simulink model "nmr_marginal_osc"  (R2025b)
settings: Solver=ode45  StartTime=0.0  StopTime=P.Tstop  MaxStep=P.maxStep  RelTol=1e-5
PreLoadFcn:
  | nmr_params
InitFcn:
  | nmr_params
undefined symbols (not defined in the file or in its folder): P
libraries: simulink x2
settings Model: Creator=paul  LastModifiedBy=paul

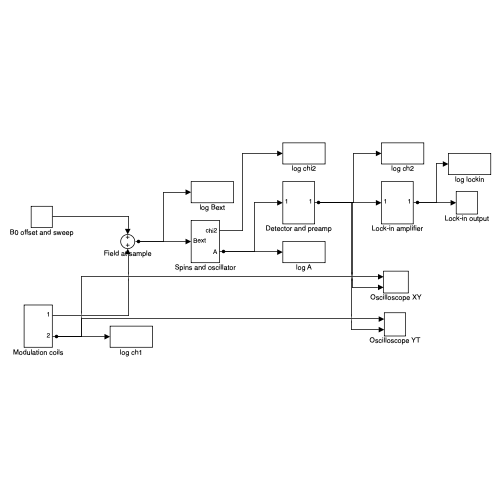
[thumbnail: Simulink's stored preview of the top-level diagram]
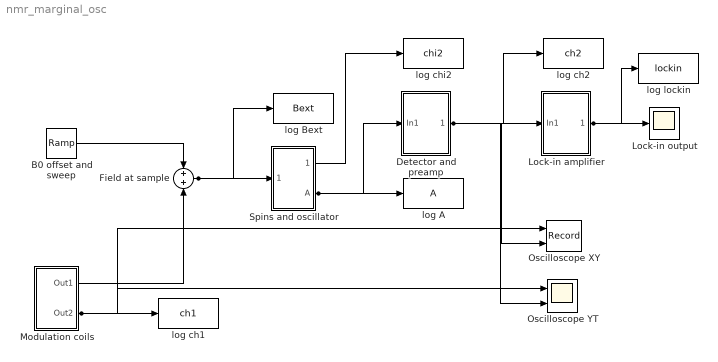
== system nmr_marginal_osc ==
  B0 offset and sweep : simulink/Sources/Ramp  slope=P.sweep  start=0  InitialOutput=P.Boff
  Detector and preamp : Subsystem
  Field at sample : Sum
  Lock-in amplifier : Subsystem
  Lock-in output : Scope
  Modulation coils : Subsystem
  Oscilloscope XY : Record  NumPorts=2.0  FileSettingsInternal="{\"entries\":[{\"content\":{\"excelSettings\":{\"content\":{},\"type\":\"Streamout.ExcelSettings\"},\"parquetSettings\":{\"content\":{},\"type\":\"Streamout.ParquetSettings\"}},\"type\":\"Streamout.FileSettingStorage\",\"uuid\":\"\"}],\"packageUris\":[\"http:\\/\\/schema.mathworks.com\\/mf0\\/streamout_blocks\\/R2020a\"],\"version\":\"1.0\"}"  FrameSettings=[0, 0]  Layout=[1 1]  SignalsInternal="{\"entries\":[{\"content\":{\"signals\":[{\"content\":{\"blockPath\":[],\"dimensions\":[1],\"domain\":\"\",\"lineColor\":\"#a2142f\",\"plots\":[ 1 ],\"port\":1,\"signalID\":1,\"signalName\":\"XY Graph:1\"},\"type\":\"RecordBlkView.Signal\",\"uuid\":\"\"},{\"content\":{\"blockPath\":[],\"dimensions\":[1],\"domain\":\"\",\"lineColor\":\"#139fff\",\"plots\":[ 1 ],\"port\":2,\"signalID\":2,\"signalName\":\"XY Graph:2\"},\"type\":\"RecordBlkView.Signal\",\"uuid\":\"\"}]},\"type\":\"RecordBlkView.InputSignals\",\"uuid\":\"\"}],\"packageUris\":[\"http:\\/\\/schema.mathworks.com\\/mf0\\/streamout_blocks\\/R2020a\"],\"version\":\"1.0\"}"  VisualizationBindings="{\"xyplotplugin\":{\"info\":[{\"series\":[{\"bindingParametersList\":[{\"parameter\":\"X-Axis\",\"signalID\":1,\"signalName\":\"XY Graph:1\"},{\"parameter\":\"Y-Axis\",\"signalID\":2,\"signalName\":\"XY Graph:2\"}],\"seriesID\":0}],\"subplotID\":1}]}}"  CompatibilityTag=XY
  Oscilloscope YT : Scope  NumInputPorts=2
  Spins and oscillator : Subsystem
  log A : ToWorkspace  VariableName=A  SaveFormat=Timeseries  SampleTime=-1
  log Bext : ToWorkspace  VariableName=Bext  SaveFormat=Timeseries  SampleTime=-1
  log ch1 : ToWorkspace  VariableName=ch1  SaveFormat=Timeseries  SampleTime=-1
  log ch2 : ToWorkspace  VariableName=ch2  SaveFormat=Timeseries  SampleTime=-1
  log chi2 : ToWorkspace  VariableName=chi2  SaveFormat=Timeseries  SampleTime=-1
  log lockin : ToWorkspace  VariableName=lockin  SaveFormat=Timeseries  SampleTime=-1
  wires:
  Lock-in amplifier/1(Out1) -> Lock-in output/1, log lockin/1
  Spins and oscillator/2(A) -> Detector and preamp/1(In1), log A/1
  Spins and oscillator/1(chi2) -> log chi2/1
  Field at sample/1 -> Spins and oscillator/1(Bext), log Bext/1
  Detector and preamp/1(Out1) -> log ch2/1, Oscilloscope XY/2, Oscilloscope YT/2, Lock-in amplifier/1(In1)
  Modulation coils/1(Out1) -> Field at sample/2
  Modulation coils/2(Out2) -> log ch1/1, Oscilloscope XY/1, Oscilloscope YT/1
  B0 offset and sweep/1 -> Field at sample/1

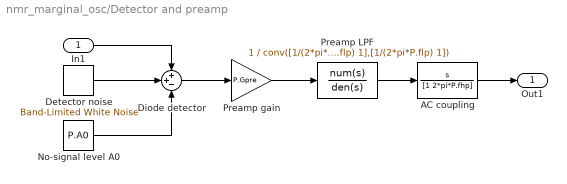
== system nmr_marginal_osc/Detector and preamp ==
  In1 : Inport
  AC coupling : TransferFcn  Numerator=[1 0]  Denominator=[1 2*pi*P.fhp]
  Detector noise : simulink/Sources/Band-Limited White Noise  Cov=P.noisePower  Ts=P.Tsn  seed=23341
  Diode detector : Sum  Inputs=++-
  No-signal level A0 : Constant  Value=P.A0
  Preamp LPF : TransferFcn  Numerator=1  Denominator=conv([1/(2*pi*P.flp) 1],[1/(2*pi*P.flp) 1])
  Preamp gain : Gain  Gain=P.Gpre
  Out1 : Outport
  wires:
  AC coupling/1 -> Out1/1
  Preamp LPF/1 -> AC coupling/1
  Preamp gain/1 -> Preamp LPF/1
  Diode detector/1 -> Preamp gain/1
  Detector noise/1 -> Diode detector/2
  No-signal level A0/1 -> Diode detector/3
  In1/1 -> Diode detector/1

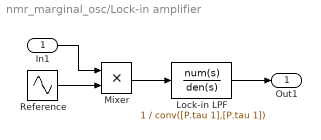
== system nmr_marginal_osc/Lock-in amplifier ==
  In1 : Inport
  Lock-in LPF : TransferFcn  Numerator=1  Denominator=conv([P.tau 1],[P.tau 1])
  Mixer : Product
  Reference : Sin  Amplitude=2  Frequency=2*pi*P.fm  Phase=-P.phi  SampleTime=0
  Out1 : Outport
  wires:
  Lock-in LPF/1 -> Out1/1
  Mixer/1 -> Lock-in LPF/1
  Reference/1 -> Mixer/2
  In1/1 -> Mixer/1

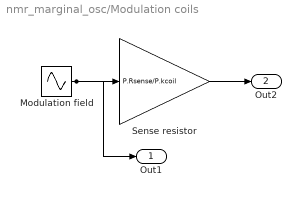
== system nmr_marginal_osc/Modulation coils ==
  Modulation field : Sin  Amplitude=P.Bmod  Frequency=2*pi*P.fm  SampleTime=0
  Sense resistor : Gain  Gain=P.Rsense/P.kcoil
  Out1 : Outport
  Out2 : Outport  Port=2
  wires:
  Sense resistor/1 -> Out2/1
  Modulation field/1 -> Out1/1, Sense resistor/1

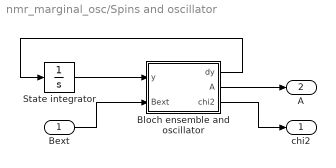
== system nmr_marginal_osc/Spins and oscillator ==
  Bext : Inport
  Bloch ensemble and oscillator : MATLAB Function  TreatAsAtomicUnit=on
  State integrator : Integrator  InitialCondition=P.y0
  chi2 : Outport
  A : Outport  Port=2
  wires:
  Bloch ensemble and oscillator/3(chi2) -> chi2/1
  Bloch ensemble and oscillator/2(A) -> A/1
  Bext/1 -> Bloch ensemble and oscillator/2(Bext)
  Bloch ensemble and oscillator/1(dy) -> State integrator/1
  State integrator/1 -> Bloch ensemble and oscillator/1(y)

== matlab function nmr_marginal_osc/Spins and oscillator/Bloch ensemble and oscillator ==
  data: y input; dy output; Bext input; A output; chi2 output; P parameter
function [dy, A, chi2] = spins_osc(y, Bext, P)
% Rotating-frame Bloch equations for an isochromat ensemble, coupled to
% the averaged amplitude A of a marginal oscillator.
N  = numel(P.dB);
Mx = y(1:N); My = y(N+1:2*N); Mz = y(2*N+1:3*N);
A  = max(y(end), 1e-9);
D  = P.gamma*(P.Bres + Bext + P.dB) - P.w0;   % offsets, rad/s
w1 = P.gamma*P.kB1*A;                         % RF nutation rate
dMx = D.*My - Mx/P.T2;
dMy = -D.*Mx + w1*Mz - My/P.T2;
dMz = -w1*My - (Mz - 1)/P.T1;
chi2 = P.chi0*P.Bres*(P.wiso'*My)/(2*P.kB1*A);  % absorption chi''
dA = (P.w0/(2*P.Q0))*(P.eps - (A/P.As)^2)*A - (P.w0/2)*P.eta*chi2*A;
dy = [dMx; dMy; dMz; dA];
